simulink model "Batteries"  (R2026b)
settings: Solver=VariableStepAuto
undefined symbols (not defined in the file or in its folder): battery_builder_rtmsupport, gcbh
libraries: Batteries_lib x10
settings Model: Creator=andrei  LastModifiedBy=andrei

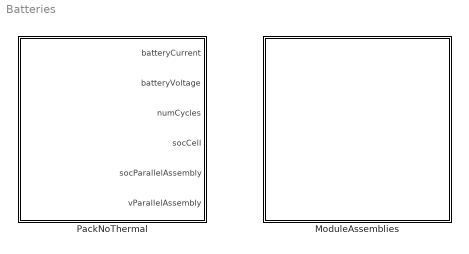
== system Batteries ==
  ModuleAssemblies : Subsystem
  PackNoThermal : Subsystem  LoadFcn=battery_builder_rtmsupport('loadfcn',gcbh);
      settings: CopyFcn=battery_builder_rtmsupport('copyfcn',gcbh);  PreCopyFcn=battery_builder_rtmsupport('precopyfcn',gcbh);  PreDeleteFcn=battery_builder_rtmsupport('predeletefcn',gcbh);  PortSchema="{\"entries\":[{\"content\":{\"sides\":[{\"content\":{\"connectorIds\":[\"LConn1\"]},\"type\":\"ConnectorPlacement.EquallySpacedRectSide\",\"uuid\":\"dcefa4cb-5347-4db9-a4bb-b951e3d91390\"},{\"content\":{\"connectorIds\":[\"RConn1\"],\"side\":\"RIGHT\"},\"type\":\"ConnectorPlacement.EquallySpacedRectSide\",\"uuid\":\"aeb17dee-f2a5-4d63-887b-6da27d52d7b7\"},{\"content\":{\"side\":\"TOP\"},\"type\":\"ConnectorPlacement.EquallySpacedRectSide\",\"uuid\":\"cfb96706-c05e-4745-bfe0-c570812fde5c\"},{\"content\":{\"connectorIds\":[\"Out1\",\"Out2\",\"Out3\",\"Out4\",\"Out5\",\"Out6\"],\"side\":\"BOTTOM\"},\"type\":\"ConnectorPlacement.EquallySpacedRectSide\",\"uuid\":\"433bdf42-6f85-4686-85d7-f0461854e351\"}]},\"type\":\"ConnectorPlacement.EquallySpacedConnector\",\"uuid\":\"fe86a992-77e4-407d-ab55-7155ee49e73e\"}],\"packageUris\":[\"http://schema.mathworks.com/mf0/Connector/R2020b\"],\"version\":\"1.0\"}"
      mask Display: image('$imagefile')

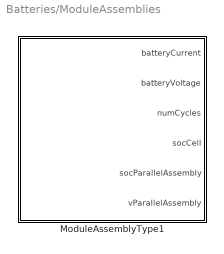
== system Batteries/ModuleAssemblies ==
  ModuleAssemblyType1 : Subsystem  LoadFcn=battery_builder_rtmsupport('loadfcn',gcbh);
      settings: CopyFcn=battery_builder_rtmsupport('copyfcn',gcbh);  PreCopyFcn=battery_builder_rtmsupport('precopyfcn',gcbh);  PreDeleteFcn=battery_builder_rtmsupport('predeletefcn',gcbh);  PortSchema="{\"entries\":[{\"content\":{\"sides\":[{\"content\":{\"connectorIds\":[\"LConn1\"]},\"type\":\"ConnectorPlacement.EquallySpacedRectSide\",\"uuid\":\"dcefa4cb-5347-4db9-a4bb-b951e3d91390\"},{\"content\":{\"connectorIds\":[\"RConn1\"],\"side\":\"RIGHT\"},\"type\":\"ConnectorPlacement.EquallySpacedRectSide\",\"uuid\":\"aeb17dee-f2a5-4d63-887b-6da27d52d7b7\"},{\"content\":{\"side\":\"TOP\"},\"type\":\"ConnectorPlacement.EquallySpacedRectSide\",\"uuid\":\"cfb96706-c05e-4745-bfe0-c570812fde5c\"},{\"content\":{\"connectorIds\":[\"Out1\",\"Out2\",\"Out3\",\"Out4\",\"Out5\",\"Out6\"],\"side\":\"BOTTOM\"},\"type\":\"ConnectorPlacement.EquallySpacedRectSide\",\"uuid\":\"431ac705-a0e6-4cbc-989d-1f8ff93ff9b4\"}]},\"type\":\"ConnectorPlacement.EquallySpacedConnector\",\"uuid\":\"fe86a992-77e4-407d-ab55-7155ee49e73e\"}],\"packageUris\":[\"http://schema.mathworks.com/mf0/Connector/R2020b\"],\"version\":\"1.0\"}"
      mask Display: image('$imagefile')

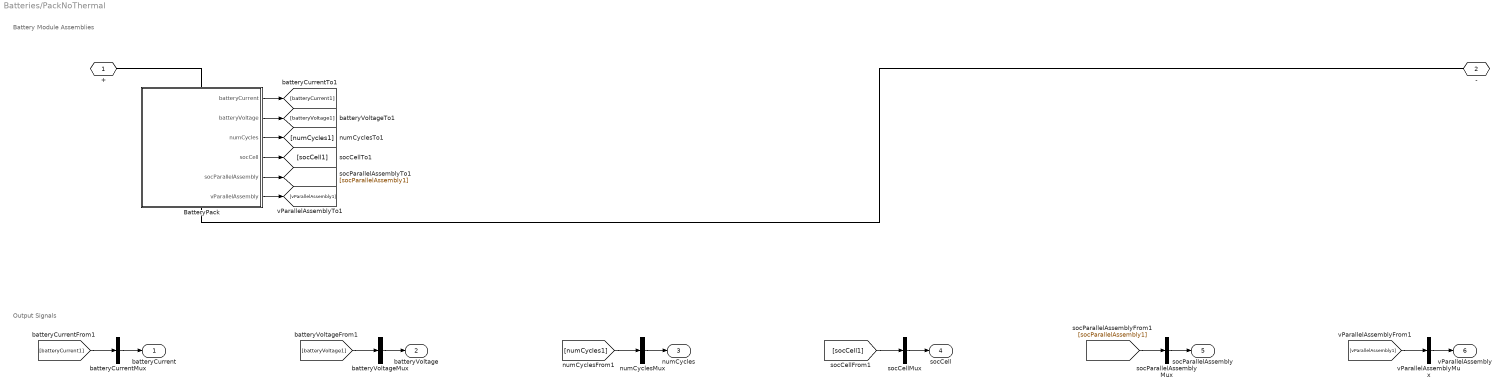
== system Batteries/PackNoThermal ==
  note: Battery Module Assemblies
  note: Output Signals
  BatteryPack : Subsystem  LoadFcn=battery_builder_rtmsupport('loadfcn',gcbh);
      settings: CopyFcn=battery_builder_rtmsupport('copyfcn',gcbh);  PreCopyFcn=battery_builder_rtmsupport('precopyfcn',gcbh);  PreDeleteFcn=battery_builder_rtmsupport('predeletefcn',gcbh);  PortSchema="{\"entries\":[{\"content\":{\"sides\":[{\"content\":{\"connectorIds\":[\"LConn1\"]},\"type\":\"ConnectorPlacement.EquallySpacedRectSide\",\"uuid\":\"dcefa4cb-5347-4db9-a4bb-b951e3d91390\"},{\"content\":{\"connectorIds\":[\"RConn1\"],\"side\":\"RIGHT\"},\"type\":\"ConnectorPlacement.EquallySpacedRectSide\",\"uuid\":\"aeb17dee-f2a5-4d63-887b-6da27d52d7b7\"},{\"content\":{\"side\":\"TOP\"},\"type\":\"ConnectorPlacement.EquallySpacedRectSide\",\"uuid\":\"cfb96706-c05e-4745-bfe0-c570812fde5c\"},{\"content\":{\"connectorIds\":[\"Out1\",\"Out2\",\"Out3\",\"Out4\",\"Out5\",\"Out6\"],\"side\":\"BOTTOM\"},\"type\":\"ConnectorPlacement.EquallySpacedRectSide\",\"uuid\":\"431ac705-a0e6-4cbc-989d-1f8ff93ff9b4\"}]},\"type\":\"ConnectorPlacement.EquallySpacedConnector\",\"uuid\":\"fe86a992-77e4-407d-ab55-7155ee49e73e\"}],\"packageUris\":[\"http://schema.mathworks.com/mf0/Connector/R2020b\"],\"version\":\"1.0\"}"
      mask Display: image('$imagefile')
  batteryCurrentMux : Mux  Inputs=1
  batteryVoltageMux : Mux  Inputs=1
  numCyclesMux : Mux  Inputs=1
  socCellMux : Mux  Inputs=1
  socParallelAssemblyMux : Mux  Inputs=1
  vParallelAssemblyMux : Mux  Inputs=1
  + : PMIOPort  Side=Left
  - : PMIOPort  Port=2  Side=Right
  batteryCurrent : Outport
  batteryVoltage : Outport  Port=2
  numCycles : Outport  Port=3
  socCell : Outport  Port=4
  socParallelAssembly : Outport  Port=5
  vParallelAssembly : Outport  Port=6
  wires:
  BatteryPack/1(batteryCurrent) -> [batteryCurrent1]
  batteryCurrentMux/1 -> batteryCurrent/1
  [batteryCurrent1] -> batteryCurrentMux/1
  BatteryPack/2(batteryVoltage) -> [batteryVoltage1]
  batteryVoltageMux/1 -> batteryVoltage/1
  [batteryVoltage1] -> batteryVoltageMux/1
  BatteryPack/3(numCycles) -> [numCycles1]
  numCyclesMux/1 -> numCycles/1
  [numCycles1] -> numCyclesMux/1
  BatteryPack/4(socCell) -> [socCell1]
  socCellMux/1 -> socCell/1
  [socCell1] -> socCellMux/1
  BatteryPack/5(socParallelAssembly) -> [socParallelAssembly1]
  socParallelAssemblyMux/1 -> socParallelAssembly/1
  [socParallelAssembly1] -> socParallelAssemblyMux/1
  BatteryPack/6(vParallelAssembly) -> [vParallelAssembly1]
  vParallelAssemblyMux/1 -> vParallelAssembly/1
  [vParallelAssembly1] -> vParallelAssemblyMux/1
  connections:
  BatteryPack/LConn1 -- +/RConn1
  BatteryPack/RConn1 -- -/RConn1

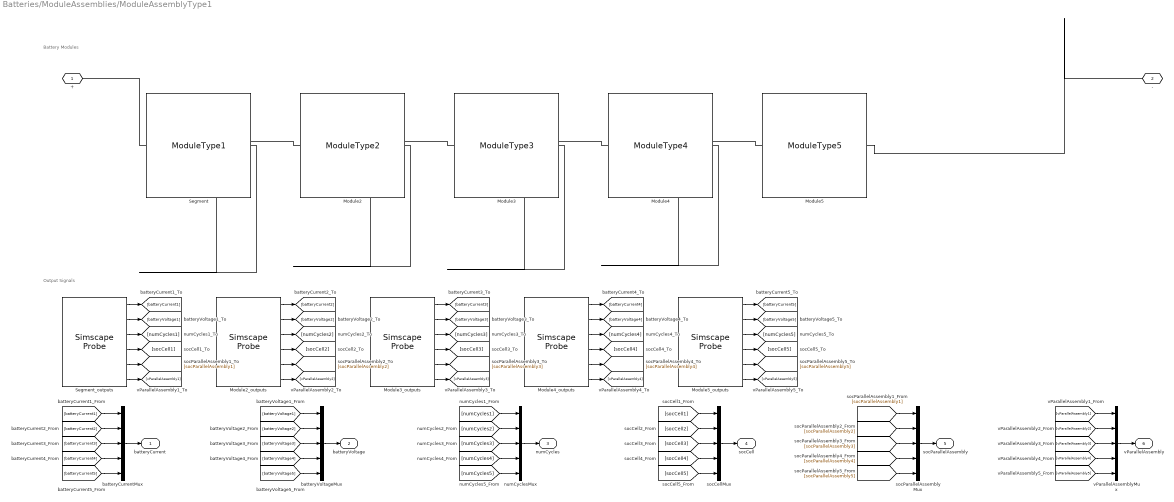
== system Batteries/ModuleAssemblies/ModuleAssemblyType1 ==
  note: Battery Modules
  note: Output Signals
  Module2 : Batteries_lib/Modules/ModuleType2  BatteryCapacityCell=27 A*hr  ExtrapolationMethodCell=simscape.enum.extrapolation.nearest  SOCBreakpointsCell=[0, .1, .25, .5, .75, .9, 1]  TemperatureBreakpointsCell=[278, 293, 313] K  OpenCircuitVoltageThermalCell=[3.49, 3.5, 3.51; 3.55, 3.57, 3.56; 3.62, 3.63, 3.64; 3.71, 3.71, 3.72; 3.91, 3.93, 3.94; 4.07, 4.08, 4.08; 4.19, 4.19, 4.19] V  VoltageRangeCell=[0, inf] V  ResistanceSOCBreakpointsCell=[0, .1, .25, .5, .75, .9, 1]  ResistanceTemperatureBreakpointsCell=[278, 293, 313] K  R0ThermalCell=[.0117, .0085, .009; .011, .0085, .009; .0114, .0087, .0092; .0107, .0082, .0088; .0107, .0083, .0091; .0113, .0085, .0089; .0116, .0085, .0089] Ohm  SimulationTemperatureCell=298.15 K  socCell_specify=off  socCell_priority=High  socCell=repmat(1, 75, 1)  socCell_nominal_specify=off  socCell_nominal_value=1  socCell_nominal_unit=1  batteryVoltage_specify=off  batteryVoltage_priority=None  batteryVoltage=repmat(0, 75, 1) V  batteryVoltage_nominal_specify=off  batteryVoltage_nominal_value=1  batteryVoltage_nominal_unit=V  batteryCurrent_specify=off  batteryCurrent_priority=None  batteryCurrent=repmat(0, 75, 1) A  batteryCurrent_nominal_specify=off  batteryCurrent_nominal_value=1  batteryCurrent_nominal_unit=A  numCycles_specify=off  numCycles_priority=High  numCycles=repmat(0, 75, 1)  numCycles_nominal_specify=off  numCycles_nominal_value=1  numCycles_nominal_unit=1  vParallelAssembly_specify=off  vParallelAssembly_priority=None  vParallelAssembly=repmat(0, 15, 1) V  vParallelAssembly_nominal_specify=off  vParallelAssembly_nominal_value=1  vParallelAssembly_nominal_unit=V  socParallelAssembly_specify=off  socParallelAssembly_priority=None  socParallelAssembly=repmat(1, 15, 1)  socParallelAssembly_nominal_specify=off  socParallelAssembly_nominal_value=1  socParallelAssembly_nominal_unit=1
  Module2_outputs : SimscapeProbe  BoundBlock=4  Variables="{\"batteryCurrent\":{\"Probing\":\"ON\"},\"batteryVoltage\":{\"Probing\":\"ON\"},\"numCycles\":{\"Probing\":\"ON\"},\"socCell\":{\"Probing\":\"ON\"},\"socParallelAssembly\":{\"Probing\":\"ON\"},\"vParallelAssembly\":{\"Probing\":\"ON\"}}"
  Module3 : Batteries_lib/Modules/ModuleType3  BatteryCapacityCell=27 A*hr  ExtrapolationMethodCell=simscape.enum.extrapolation.nearest  SOCBreakpointsCell=[0, .1, .25, .5, .75, .9, 1]  TemperatureBreakpointsCell=[278, 293, 313] K  OpenCircuitVoltageThermalCell=[3.49, 3.5, 3.51; 3.55, 3.57, 3.56; 3.62, 3.63, 3.64; 3.71, 3.71, 3.72; 3.91, 3.93, 3.94; 4.07, 4.08, 4.08; 4.19, 4.19, 4.19] V  VoltageRangeCell=[0, inf] V  ResistanceSOCBreakpointsCell=[0, .1, .25, .5, .75, .9, 1]  ResistanceTemperatureBreakpointsCell=[278, 293, 313] K  R0ThermalCell=[.0117, .0085, .009; .011, .0085, .009; .0114, .0087, .0092; .0107, .0082, .0088; .0107, .0083, .0091; .0113, .0085, .0089; .0116, .0085, .0089] Ohm  SimulationTemperatureCell=298.15 K  socCell_specify=off  socCell_priority=High  socCell=repmat(1, 75, 1)  socCell_nominal_specify=off  socCell_nominal_value=1  socCell_nominal_unit=1  batteryVoltage_specify=off  batteryVoltage_priority=None  batteryVoltage=repmat(0, 75, 1) V  batteryVoltage_nominal_specify=off  batteryVoltage_nominal_value=1  batteryVoltage_nominal_unit=V  batteryCurrent_specify=off  batteryCurrent_priority=None  batteryCurrent=repmat(0, 75, 1) A  batteryCurrent_nominal_specify=off  batteryCurrent_nominal_value=1  batteryCurrent_nominal_unit=A  numCycles_specify=off  numCycles_priority=High  numCycles=repmat(0, 75, 1)  numCycles_nominal_specify=off  numCycles_nominal_value=1  numCycles_nominal_unit=1  vParallelAssembly_specify=off  vParallelAssembly_priority=None  vParallelAssembly=repmat(0, 15, 1) V  vParallelAssembly_nominal_specify=off  vParallelAssembly_nominal_value=1  vParallelAssembly_nominal_unit=V  socParallelAssembly_specify=off  socParallelAssembly_priority=None  socParallelAssembly=repmat(1, 15, 1)  socParallelAssembly_nominal_specify=off  socParallelAssembly_nominal_value=1  socParallelAssembly_nominal_unit=1
  Module3_outputs : SimscapeProbe  BoundBlock=5  Variables="{\"batteryCurrent\":{\"Probing\":\"ON\"},\"batteryVoltage\":{\"Probing\":\"ON\"},\"numCycles\":{\"Probing\":\"ON\"},\"socCell\":{\"Probing\":\"ON\"},\"socParallelAssembly\":{\"Probing\":\"ON\"},\"vParallelAssembly\":{\"Probing\":\"ON\"}}"
  Module4 : Batteries_lib/Modules/ModuleType4  BatteryCapacityCell=27 A*hr  ExtrapolationMethodCell=simscape.enum.extrapolation.nearest  SOCBreakpointsCell=[0, .1, .25, .5, .75, .9, 1]  TemperatureBreakpointsCell=[278, 293, 313] K  OpenCircuitVoltageThermalCell=[3.49, 3.5, 3.51; 3.55, 3.57, 3.56; 3.62, 3.63, 3.64; 3.71, 3.71, 3.72; 3.91, 3.93, 3.94; 4.07, 4.08, 4.08; 4.19, 4.19, 4.19] V  VoltageRangeCell=[0, inf] V  ResistanceSOCBreakpointsCell=[0, .1, .25, .5, .75, .9, 1]  ResistanceTemperatureBreakpointsCell=[278, 293, 313] K  R0ThermalCell=[.0117, .0085, .009; .011, .0085, .009; .0114, .0087, .0092; .0107, .0082, .0088; .0107, .0083, .0091; .0113, .0085, .0089; .0116, .0085, .0089] Ohm  SimulationTemperatureCell=298.15 K  socCell_specify=off  socCell_priority=High  socCell=repmat(1, 75, 1)  socCell_nominal_specify=off  socCell_nominal_value=1  socCell_nominal_unit=1  batteryVoltage_specify=off  batteryVoltage_priority=None  batteryVoltage=repmat(0, 75, 1) V  batteryVoltage_nominal_specify=off  batteryVoltage_nominal_value=1  batteryVoltage_nominal_unit=V  batteryCurrent_specify=off  batteryCurrent_priority=None  batteryCurrent=repmat(0, 75, 1) A  batteryCurrent_nominal_specify=off  batteryCurrent_nominal_value=1  batteryCurrent_nominal_unit=A  numCycles_specify=off  numCycles_priority=High  numCycles=repmat(0, 75, 1)  numCycles_nominal_specify=off  numCycles_nominal_value=1  numCycles_nominal_unit=1  vParallelAssembly_specify=off  vParallelAssembly_priority=None  vParallelAssembly=repmat(0, 15, 1) V  vParallelAssembly_nominal_specify=off  vParallelAssembly_nominal_value=1  vParallelAssembly_nominal_unit=V  socParallelAssembly_specify=off  socParallelAssembly_priority=None  socParallelAssembly=repmat(1, 15, 1)  socParallelAssembly_nominal_specify=off  socParallelAssembly_nominal_value=1  socParallelAssembly_nominal_unit=1
  Module4_outputs : SimscapeProbe  BoundBlock=6  Variables="{\"batteryCurrent\":{\"Probing\":\"ON\"},\"batteryVoltage\":{\"Probing\":\"ON\"},\"numCycles\":{\"Probing\":\"ON\"},\"socCell\":{\"Probing\":\"ON\"},\"socParallelAssembly\":{\"Probing\":\"ON\"},\"vParallelAssembly\":{\"Probing\":\"ON\"}}"
  Module5 : Batteries_lib/Modules/ModuleType5  BatteryCapacityCell=27 A*hr  ExtrapolationMethodCell=simscape.enum.extrapolation.nearest  SOCBreakpointsCell=[0, .1, .25, .5, .75, .9, 1]  TemperatureBreakpointsCell=[278, 293, 313] K  OpenCircuitVoltageThermalCell=[3.49, 3.5, 3.51; 3.55, 3.57, 3.56; 3.62, 3.63, 3.64; 3.71, 3.71, 3.72; 3.91, 3.93, 3.94; 4.07, 4.08, 4.08; 4.19, 4.19, 4.19] V  VoltageRangeCell=[0, inf] V  ResistanceSOCBreakpointsCell=[0, .1, .25, .5, .75, .9, 1]  ResistanceTemperatureBreakpointsCell=[278, 293, 313] K  R0ThermalCell=[.0117, .0085, .009; .011, .0085, .009; .0114, .0087, .0092; .0107, .0082, .0088; .0107, .0083, .0091; .0113, .0085, .0089; .0116, .0085, .0089] Ohm  SimulationTemperatureCell=298.15 K  socCell_specify=off  socCell_priority=High  socCell=repmat(1, 75, 1)  socCell_nominal_specify=off  socCell_nominal_value=1  socCell_nominal_unit=1  batteryVoltage_specify=off  batteryVoltage_priority=None  batteryVoltage=repmat(0, 75, 1) V  batteryVoltage_nominal_specify=off  batteryVoltage_nominal_value=1  batteryVoltage_nominal_unit=V  batteryCurrent_specify=off  batteryCurrent_priority=None  batteryCurrent=repmat(0, 75, 1) A  batteryCurrent_nominal_specify=off  batteryCurrent_nominal_value=1  batteryCurrent_nominal_unit=A  numCycles_specify=off  numCycles_priority=High  numCycles=repmat(0, 75, 1)  numCycles_nominal_specify=off  numCycles_nominal_value=1  numCycles_nominal_unit=1  vParallelAssembly_specify=off  vParallelAssembly_priority=None  vParallelAssembly=repmat(0, 15, 1) V  vParallelAssembly_nominal_specify=off  vParallelAssembly_nominal_value=1  vParallelAssembly_nominal_unit=V  socParallelAssembly_specify=off  socParallelAssembly_priority=None  socParallelAssembly=repmat(1, 15, 1)  socParallelAssembly_nominal_specify=off  socParallelAssembly_nominal_value=1  socParallelAssembly_nominal_unit=1
  Module5_outputs : SimscapeProbe  BoundBlock=7  Variables="{\"batteryCurrent\":{\"Probing\":\"ON\"},\"batteryVoltage\":{\"Probing\":\"ON\"},\"numCycles\":{\"Probing\":\"ON\"},\"socCell\":{\"Probing\":\"ON\"},\"socParallelAssembly\":{\"Probing\":\"ON\"},\"vParallelAssembly\":{\"Probing\":\"ON\"}}"
  Segment : Batteries_lib/Modules/ModuleType1  BatteryCapacityCell=27 A*hr  ExtrapolationMethodCell=simscape.enum.extrapolation.nearest  SOCBreakpointsCell=[0, .1, .25, .5, .75, .9, 1]  TemperatureBreakpointsCell=[278, 293, 313] K  OpenCircuitVoltageThermalCell=[3.49, 3.5, 3.51; 3.55, 3.57, 3.56; 3.62, 3.63, 3.64; 3.71, 3.71, 3.72; 3.91, 3.93, 3.94; 4.07, 4.08, 4.08; 4.19, 4.19, 4.19] V  VoltageRangeCell=[0, inf] V  ResistanceSOCBreakpointsCell=[0, .1, .25, .5, .75, .9, 1]  ResistanceTemperatureBreakpointsCell=[278, 293, 313] K  R0ThermalCell=[.0117, .0085, .009; .011, .0085, .009; .0114, .0087, .0092; .0107, .0082, .0088; .0107, .0083, .0091; .0113, .0085, .0089; .0116, .0085, .0089] Ohm  SimulationTemperatureCell=298.15 K  socCell_specify=off  socCell_priority=High  socCell=repmat(1, 75, 1)  socCell_nominal_specify=off  socCell_nominal_value=1  socCell_nominal_unit=1  batteryVoltage_specify=off  batteryVoltage_priority=None  batteryVoltage=repmat(0, 75, 1) V  batteryVoltage_nominal_specify=off  batteryVoltage_nominal_value=1  batteryVoltage_nominal_unit=V  batteryCurrent_specify=off  batteryCurrent_priority=None  batteryCurrent=repmat(0, 75, 1) A  batteryCurrent_nominal_specify=off  batteryCurrent_nominal_value=1  batteryCurrent_nominal_unit=A  numCycles_specify=off  numCycles_priority=High  numCycles=repmat(0, 75, 1)  numCycles_nominal_specify=off  numCycles_nominal_value=1  numCycles_nominal_unit=1  vParallelAssembly_specify=off  vParallelAssembly_priority=None  vParallelAssembly=repmat(0, 15, 1) V  vParallelAssembly_nominal_specify=off  vParallelAssembly_nominal_value=1  vParallelAssembly_nominal_unit=V  socParallelAssembly_specify=off  socParallelAssembly_priority=None  socParallelAssembly=repmat(1, 15, 1)  socParallelAssembly_nominal_specify=off  socParallelAssembly_nominal_value=1  socParallelAssembly_nominal_unit=1
  Segment_outputs : SimscapeProbe  BoundBlock=3  Variables="{\"batteryCurrent\":{\"Probing\":\"ON\"},\"batteryVoltage\":{\"Probing\":\"ON\"},\"numCycles\":{\"Probing\":\"ON\"},\"socCell\":{\"Probing\":\"ON\"},\"socParallelAssembly\":{\"Probing\":\"ON\"},\"vParallelAssembly\":{\"Probing\":\"ON\"}}"
  batteryCurrentMux : Mux  Inputs=5
  batteryVoltageMux : Mux  Inputs=5
  numCyclesMux : Mux  Inputs=5
  socCellMux : Mux  Inputs=5
  socParallelAssemblyMux : Mux  Inputs=5
  vParallelAssemblyMux : Mux  Inputs=5
  + : PMIOPort  Side=Left
  - : PMIOPort  Port=2  Side=Right
  batteryCurrent : Outport
  batteryVoltage : Outport  Port=2
  numCycles : Outport  Port=3
  socCell : Outport  Port=4
  socParallelAssembly : Outport  Port=5
  vParallelAssembly : Outport  Port=6
  wires:
  Segment_outputs/1 -> [batteryCurrent1]
  batteryCurrentMux/1 -> batteryCurrent/1
  [batteryCurrent1] -> batteryCurrentMux/1
  Segment_outputs/2 -> [batteryVoltage1]
  batteryVoltageMux/1 -> batteryVoltage/1
  [batteryVoltage1] -> batteryVoltageMux/1
  Segment_outputs/3 -> [numCycles1]
  numCyclesMux/1 -> numCycles/1
  [numCycles1] -> numCyclesMux/1
  Segment_outputs/4 -> [socCell1]
  socCellMux/1 -> socCell/1
  [socCell1] -> socCellMux/1
  Segment_outputs/5 -> [socParallelAssembly1]
  socParallelAssemblyMux/1 -> socParallelAssembly/1
  [socParallelAssembly1] -> socParallelAssemblyMux/1
  Segment_outputs/6 -> [vParallelAssembly1]
  vParallelAssemblyMux/1 -> vParallelAssembly/1
  [vParallelAssembly1] -> vParallelAssemblyMux/1
  Module2_outputs/1 -> [batteryCurrent2]
  [batteryCurrent2] -> batteryCurrentMux/2
  Module2_outputs/2 -> [batteryVoltage2]
  [batteryVoltage2] -> batteryVoltageMux/2
  Module2_outputs/3 -> [numCycles2]
  [numCycles2] -> numCyclesMux/2
  Module2_outputs/4 -> [socCell2]
  [socCell2] -> socCellMux/2
  Module2_outputs/5 -> [socParallelAssembly2]
  [socParallelAssembly2] -> socParallelAssemblyMux/2
  Module2_outputs/6 -> [vParallelAssembly2]
  [vParallelAssembly2] -> vParallelAssemblyMux/2
  Module3_outputs/1 -> [batteryCurrent3]
  [batteryCurrent3] -> batteryCurrentMux/3
  Module3_outputs/2 -> [batteryVoltage3]
  [batteryVoltage3] -> batteryVoltageMux/3
  Module3_outputs/3 -> [numCycles3]
  [numCycles3] -> numCyclesMux/3
  Module3_outputs/4 -> [socCell3]
  [socCell3] -> socCellMux/3
  Module3_outputs/5 -> [socParallelAssembly3]
  [socParallelAssembly3] -> socParallelAssemblyMux/3
  Module3_outputs/6 -> [vParallelAssembly3]
  [vParallelAssembly3] -> vParallelAssemblyMux/3
  Module4_outputs/1 -> [batteryCurrent4]
  [batteryCurrent4] -> batteryCurrentMux/4
  Module4_outputs/2 -> [batteryVoltage4]
  [batteryVoltage4] -> batteryVoltageMux/4
  Module4_outputs/3 -> [numCycles4]
  [numCycles4] -> numCyclesMux/4
  Module4_outputs/4 -> [socCell4]
  [socCell4] -> socCellMux/4
  Module4_outputs/5 -> [socParallelAssembly4]
  [socParallelAssembly4] -> socParallelAssemblyMux/4
  Module4_outputs/6 -> [vParallelAssembly4]
  [vParallelAssembly4] -> vParallelAssemblyMux/4
  Module5_outputs/1 -> [batteryCurrent5]
  [batteryCurrent5] -> batteryCurrentMux/5
  Module5_outputs/2 -> [batteryVoltage5]
  [batteryVoltage5] -> batteryVoltageMux/5
  Module5_outputs/3 -> [numCycles5]
  [numCycles5] -> numCyclesMux/5
  Module5_outputs/4 -> [socCell5]
  [socCell5] -> socCellMux/5
  Module5_outputs/5 -> [socParallelAssembly5]
  [socParallelAssembly5] -> socParallelAssemblyMux/5
  Module5_outputs/6 -> [vParallelAssembly5]
  [vParallelAssembly5] -> vParallelAssemblyMux/5
  connections:
  Module2/LConn1 -- Segment/RConn1
  Module3/LConn1 -- Module2/RConn1
  Module4/LConn1 -- Module3/RConn1
  Module5/LConn1 -- Module4/RConn1
  Segment/LConn1 -- +/RConn1
  Module5/RConn1 -- -/RConn1

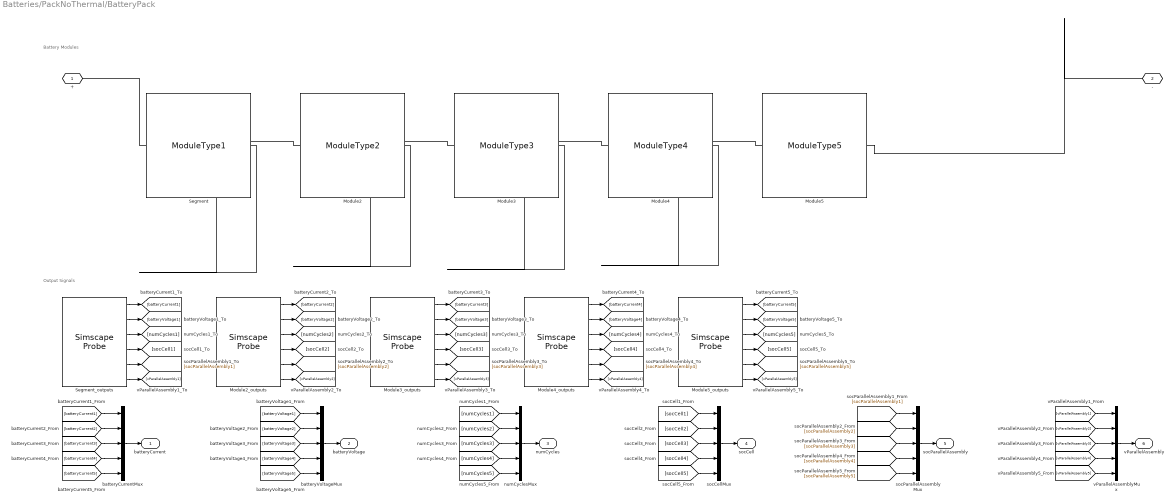
== system Batteries/PackNoThermal/BatteryPack ==
  note: Output Signals
  note: Battery Modules
  Module2 : Batteries_lib/Modules/ModuleType2  BatteryCapacityCell=BatteryPack.Segment.BatteryCapacityCell A*hr  ExtrapolationMethodCell=simscape.enum.extrapolation.nearest  SOCBreakpointsCell=BatteryPack.Segment.SOCBreakpointsCell  TemperatureBreakpointsCell=BatteryPack.Segment.TemperatureBreakpointsCell K  OpenCircuitVoltageThermalCell=BatteryPack.Segment.OpenCircuitVoltageThermalCell V  VoltageRangeCell=BatteryPack.Segment.VoltageRangeCell V  ResistanceSOCBreakpointsCell=BatteryPack.Segment.ResistanceSOCBreakpointsCell  ResistanceTemperatureBreakpointsCell=BatteryPack.Segment.ResistanceTemperatureBreakpointsCell K  R0ThermalCell=BatteryPack.Segment.R0ThermalCell Ohm  SimulationTemperatureCell=BatteryPack.Segment.SimulationTemperatureCell K  socCell_specify=on  socCell_priority=High  socCell=[1;1;1;1;1;1;1;1;1;1;1;1;1;1;1;1;1;1;1;1;1;1;1;1;1;1;1;1;1;1;1;1;1;1;1;1;1;1;1;1;1;1;1;1;1;1;1;1;1;1;1;1;1;1;1;1;1;1;1;1;1;1;1;1;1;1;1;1;1;1;1;1;1;1;1]  socCell_nominal_specify=off  socCell_nominal_value=1  socCell_nominal_unit=1  batteryVoltage_specify=on  batteryVoltage_priority=None  batteryVoltage=[0;0;0;0;0;0;0;0;0;0;0;0;0;0;0;0;0;0;0;0;0;0;0;0;0;0;0;0;0;0;0;0;0;0;0;0;0;0;0;0;0;0;0;0;0;0;0;0;0;0;0;0;0;0;0;0;0;0;0;0;0;0;0;0;0;0;0;0;0;0;0;0;0;0;0] V  batteryVoltage_nominal_specify=off  batteryVoltage_nominal_value=1  batteryVoltage_nominal_unit=V  batteryCurrent_specify=on  batteryCurrent_priority=None  batteryCurrent=[0;0;0;0;0;0;0;0;0;0;0;0;0;0;0;0;0;0;0;0;0;0;0;0;0;0;0;0;0;0;0;0;0;0;0;0;0;0;0;0;0;0;0;0;0;0;0;0;0;0;0;0;0;0;0;0;0;0;0;0;0;0;0;0;0;0;0;0;0;0;0;0;0;0;0] A  batteryCurrent_nominal_specify=off  batteryCurrent_nominal_value=1  batteryCurrent_nominal_unit=A  numCycles_specify=on  numCycles_priority=High  numCycles=[0;0;0;0;0;0;0;0;0;0;0;0;0;0;0;0;0;0;0;0;0;0;0;0;0;0;0;0;0;0;0;0;0;0;0;0;0;0;0;0;0;0;0;0;0;0;0;0;0;0;0;0;0;0;0;0;0;0;0;0;0;0;0;0;0;0;0;0;0;0;0;0;0;0;0]  numCycles_nominal_specify=off  numCycles_nominal_value=1  numCycles_nominal_unit=1  vParallelAssembly_specify=on  vParallelAssembly_priority=None  vParallelAssembly=[0;0;0;0;0;0;0;0;0;0;0;0;0;0;0] V  vParallelAssembly_nominal_specify=off  vParallelAssembly_nominal_value=1  vParallelAssembly_nominal_unit=V  socParallelAssembly_specify=on  socParallelAssembly_priority=None  socParallelAssembly=[1;1;1;1;1;1;1;1;1;1;1;1;1;1;1]  socParallelAssembly_nominal_specify=off  socParallelAssembly_nominal_value=1  socParallelAssembly_nominal_unit=1
  Module2_outputs : SimscapeProbe  BoundBlock=91  Variables="{\"batteryCurrent\":{\"Probing\":\"ON\"},\"batteryVoltage\":{\"Probing\":\"ON\"},\"numCycles\":{\"Probing\":\"ON\"},\"socCell\":{\"Probing\":\"ON\"},\"socParallelAssembly\":{\"Probing\":\"ON\"},\"vParallelAssembly\":{\"Probing\":\"ON\"}}"
  Module3 : Batteries_lib/Modules/ModuleType3  BatteryCapacityCell=BatteryPack.Segment.BatteryCapacityCell A*hr  ExtrapolationMethodCell=simscape.enum.extrapolation.nearest  SOCBreakpointsCell=BatteryPack.Segment.SOCBreakpointsCell  TemperatureBreakpointsCell=BatteryPack.Segment.TemperatureBreakpointsCell K  OpenCircuitVoltageThermalCell=BatteryPack.Segment.OpenCircuitVoltageThermalCell V  VoltageRangeCell=BatteryPack.Segment.VoltageRangeCell V  ResistanceSOCBreakpointsCell=BatteryPack.Segment.ResistanceSOCBreakpointsCell  ResistanceTemperatureBreakpointsCell=BatteryPack.Segment.ResistanceTemperatureBreakpointsCell K  R0ThermalCell=BatteryPack.Segment.R0ThermalCell Ohm  SimulationTemperatureCell=BatteryPack.Segment.SimulationTemperatureCell K  socCell_specify=on  socCell_priority=High  socCell=[1;1;1;1;1;1;1;1;1;1;1;1;1;1;1;1;1;1;1;1;1;1;1;1;1;1;1;1;1;1;1;1;1;1;1;1;1;1;1;1;1;1;1;1;1;1;1;1;1;1;1;1;1;1;1;1;1;1;1;1;1;1;1;1;1;1;1;1;1;1;1;1;1;1;1]  socCell_nominal_specify=off  socCell_nominal_value=1  socCell_nominal_unit=1  batteryVoltage_specify=on  batteryVoltage_priority=None  batteryVoltage=[0;0;0;0;0;0;0;0;0;0;0;0;0;0;0;0;0;0;0;0;0;0;0;0;0;0;0;0;0;0;0;0;0;0;0;0;0;0;0;0;0;0;0;0;0;0;0;0;0;0;0;0;0;0;0;0;0;0;0;0;0;0;0;0;0;0;0;0;0;0;0;0;0;0;0] V  batteryVoltage_nominal_specify=off  batteryVoltage_nominal_value=1  batteryVoltage_nominal_unit=V  batteryCurrent_specify=on  batteryCurrent_priority=None  batteryCurrent=[0;0;0;0;0;0;0;0;0;0;0;0;0;0;0;0;0;0;0;0;0;0;0;0;0;0;0;0;0;0;0;0;0;0;0;0;0;0;0;0;0;0;0;0;0;0;0;0;0;0;0;0;0;0;0;0;0;0;0;0;0;0;0;0;0;0;0;0;0;0;0;0;0;0;0] A  batteryCurrent_nominal_specify=off  batteryCurrent_nominal_value=1  batteryCurrent_nominal_unit=A  numCycles_specify=on  numCycles_priority=High  numCycles=[0;0;0;0;0;0;0;0;0;0;0;0;0;0;0;0;0;0;0;0;0;0;0;0;0;0;0;0;0;0;0;0;0;0;0;0;0;0;0;0;0;0;0;0;0;0;0;0;0;0;0;0;0;0;0;0;0;0;0;0;0;0;0;0;0;0;0;0;0;0;0;0;0;0;0]  numCycles_nominal_specify=off  numCycles_nominal_value=1  numCycles_nominal_unit=1  vParallelAssembly_specify=on  vParallelAssembly_priority=None  vParallelAssembly=[0;0;0;0;0;0;0;0;0;0;0;0;0;0;0] V  vParallelAssembly_nominal_specify=off  vParallelAssembly_nominal_value=1  vParallelAssembly_nominal_unit=V  socParallelAssembly_specify=on  socParallelAssembly_priority=None  socParallelAssembly=[1;1;1;1;1;1;1;1;1;1;1;1;1;1;1]  socParallelAssembly_nominal_specify=off  socParallelAssembly_nominal_value=1  socParallelAssembly_nominal_unit=1
  Module3_outputs : SimscapeProbe  BoundBlock=93  Variables="{\"batteryCurrent\":{\"Probing\":\"ON\"},\"batteryVoltage\":{\"Probing\":\"ON\"},\"numCycles\":{\"Probing\":\"ON\"},\"socCell\":{\"Probing\":\"ON\"},\"socParallelAssembly\":{\"Probing\":\"ON\"},\"vParallelAssembly\":{\"Probing\":\"ON\"}}"
  Module4 : Batteries_lib/Modules/ModuleType4  BatteryCapacityCell=BatteryPack.Segment.BatteryCapacityCell A*hr  ExtrapolationMethodCell=simscape.enum.extrapolation.nearest  SOCBreakpointsCell=BatteryPack.Segment.SOCBreakpointsCell  TemperatureBreakpointsCell=BatteryPack.Segment.TemperatureBreakpointsCell K  OpenCircuitVoltageThermalCell=BatteryPack.Segment.OpenCircuitVoltageThermalCell V  VoltageRangeCell=BatteryPack.Segment.VoltageRangeCell V  ResistanceSOCBreakpointsCell=BatteryPack.Segment.ResistanceSOCBreakpointsCell  ResistanceTemperatureBreakpointsCell=BatteryPack.Segment.ResistanceTemperatureBreakpointsCell K  R0ThermalCell=BatteryPack.Segment.R0ThermalCell Ohm  SimulationTemperatureCell=BatteryPack.Segment.SimulationTemperatureCell K  socCell_specify=on  socCell_priority=High  socCell=[1;1;1;1;1;1;1;1;1;1;1;1;1;1;1;1;1;1;1;1;1;1;1;1;1;1;1;1;1;1;1;1;1;1;1;1;1;1;1;1;1;1;1;1;1;1;1;1;1;1;1;1;1;1;1;1;1;1;1;1;1;1;1;1;1;1;1;1;1;1;1;1;1;1;1]  socCell_nominal_specify=off  socCell_nominal_value=1  socCell_nominal_unit=1  batteryVoltage_specify=on  batteryVoltage_priority=None  batteryVoltage=[0;0;0;0;0;0;0;0;0;0;0;0;0;0;0;0;0;0;0;0;0;0;0;0;0;0;0;0;0;0;0;0;0;0;0;0;0;0;0;0;0;0;0;0;0;0;0;0;0;0;0;0;0;0;0;0;0;0;0;0;0;0;0;0;0;0;0;0;0;0;0;0;0;0;0] V  batteryVoltage_nominal_specify=off  batteryVoltage_nominal_value=1  batteryVoltage_nominal_unit=V  batteryCurrent_specify=on  batteryCurrent_priority=None  batteryCurrent=[0;0;0;0;0;0;0;0;0;0;0;0;0;0;0;0;0;0;0;0;0;0;0;0;0;0;0;0;0;0;0;0;0;0;0;0;0;0;0;0;0;0;0;0;0;0;0;0;0;0;0;0;0;0;0;0;0;0;0;0;0;0;0;0;0;0;0;0;0;0;0;0;0;0;0] A  batteryCurrent_nominal_specify=off  batteryCurrent_nominal_value=1  batteryCurrent_nominal_unit=A  numCycles_specify=on  numCycles_priority=High  numCycles=[0;0;0;0;0;0;0;0;0;0;0;0;0;0;0;0;0;0;0;0;0;0;0;0;0;0;0;0;0;0;0;0;0;0;0;0;0;0;0;0;0;0;0;0;0;0;0;0;0;0;0;0;0;0;0;0;0;0;0;0;0;0;0;0;0;0;0;0;0;0;0;0;0;0;0]  numCycles_nominal_specify=off  numCycles_nominal_value=1  numCycles_nominal_unit=1  vParallelAssembly_specify=on  vParallelAssembly_priority=None  vParallelAssembly=[0;0;0;0;0;0;0;0;0;0;0;0;0;0;0] V  vParallelAssembly_nominal_specify=off  vParallelAssembly_nominal_value=1  vParallelAssembly_nominal_unit=V  socParallelAssembly_specify=on  socParallelAssembly_priority=None  socParallelAssembly=[1;1;1;1;1;1;1;1;1;1;1;1;1;1;1]  socParallelAssembly_nominal_specify=off  socParallelAssembly_nominal_value=1  socParallelAssembly_nominal_unit=1
  Module4_outputs : SimscapeProbe  BoundBlock=95  Variables="{\"batteryCurrent\":{\"Probing\":\"ON\"},\"batteryVoltage\":{\"Probing\":\"ON\"},\"numCycles\":{\"Probing\":\"ON\"},\"socCell\":{\"Probing\":\"ON\"},\"socParallelAssembly\":{\"Probing\":\"ON\"},\"vParallelAssembly\":{\"Probing\":\"ON\"}}"
  Module5 : Batteries_lib/Modules/ModuleType5  BatteryCapacityCell=BatteryPack.Segment.BatteryCapacityCell A*hr  ExtrapolationMethodCell=simscape.enum.extrapolation.nearest  SOCBreakpointsCell=BatteryPack.Segment.SOCBreakpointsCell  TemperatureBreakpointsCell=BatteryPack.Segment.TemperatureBreakpointsCell K  OpenCircuitVoltageThermalCell=BatteryPack.Segment.OpenCircuitVoltageThermalCell V  VoltageRangeCell=BatteryPack.Segment.VoltageRangeCell V  ResistanceSOCBreakpointsCell=BatteryPack.Segment.ResistanceSOCBreakpointsCell  ResistanceTemperatureBreakpointsCell=BatteryPack.Segment.ResistanceTemperatureBreakpointsCell K  R0ThermalCell=BatteryPack.Segment.R0ThermalCell Ohm  SimulationTemperatureCell=BatteryPack.Segment.SimulationTemperatureCell K  socCell_specify=on  socCell_priority=High  socCell=[1;1;1;1;1;1;1;1;1;1;1;1;1;1;1;1;1;1;1;1;1;1;1;1;1;1;1;1;1;1;1;1;1;1;1;1;1;1;1;1;1;1;1;1;1;1;1;1;1;1;1;1;1;1;1;1;1;1;1;1;1;1;1;1;1;1;1;1;1;1;1;1;1;1;1]  socCell_nominal_specify=off  socCell_nominal_value=1  socCell_nominal_unit=1  batteryVoltage_specify=on  batteryVoltage_priority=None  batteryVoltage=[0;0;0;0;0;0;0;0;0;0;0;0;0;0;0;0;0;0;0;0;0;0;0;0;0;0;0;0;0;0;0;0;0;0;0;0;0;0;0;0;0;0;0;0;0;0;0;0;0;0;0;0;0;0;0;0;0;0;0;0;0;0;0;0;0;0;0;0;0;0;0;0;0;0;0] V  batteryVoltage_nominal_specify=off  batteryVoltage_nominal_value=1  batteryVoltage_nominal_unit=V  batteryCurrent_specify=on  batteryCurrent_priority=None  batteryCurrent=[0;0;0;0;0;0;0;0;0;0;0;0;0;0;0;0;0;0;0;0;0;0;0;0;0;0;0;0;0;0;0;0;0;0;0;0;0;0;0;0;0;0;0;0;0;0;0;0;0;0;0;0;0;0;0;0;0;0;0;0;0;0;0;0;0;0;0;0;0;0;0;0;0;0;0] A  batteryCurrent_nominal_specify=off  batteryCurrent_nominal_value=1  batteryCurrent_nominal_unit=A  numCycles_specify=on  numCycles_priority=High  numCycles=[0;0;0;0;0;0;0;0;0;0;0;0;0;0;0;0;0;0;0;0;0;0;0;0;0;0;0;0;0;0;0;0;0;0;0;0;0;0;0;0;0;0;0;0;0;0;0;0;0;0;0;0;0;0;0;0;0;0;0;0;0;0;0;0;0;0;0;0;0;0;0;0;0;0;0]  numCycles_nominal_specify=off  numCycles_nominal_value=1  numCycles_nominal_unit=1  vParallelAssembly_specify=on  vParallelAssembly_priority=None  vParallelAssembly=[0;0;0;0;0;0;0;0;0;0;0;0;0;0;0] V  vParallelAssembly_nominal_specify=off  vParallelAssembly_nominal_value=1  vParallelAssembly_nominal_unit=V  socParallelAssembly_specify=on  socParallelAssembly_priority=None  socParallelAssembly=[1;1;1;1;1;1;1;1;1;1;1;1;1;1;1]  socParallelAssembly_nominal_specify=off  socParallelAssembly_nominal_value=1  socParallelAssembly_nominal_unit=1
  Module5_outputs : SimscapeProbe  BoundBlock=97  Variables="{\"batteryCurrent\":{\"Probing\":\"ON\"},\"batteryVoltage\":{\"Probing\":\"ON\"},\"numCycles\":{\"Probing\":\"ON\"},\"socCell\":{\"Probing\":\"ON\"},\"socParallelAssembly\":{\"Probing\":\"ON\"},\"vParallelAssembly\":{\"Probing\":\"ON\"}}"
  Segment : Batteries_lib/Modules/ModuleType1  BatteryCapacityCell=BatteryPack.Segment.BatteryCapacityCell A*hr  ExtrapolationMethodCell=simscape.enum.extrapolation.nearest  SOCBreakpointsCell=BatteryPack.Segment.SOCBreakpointsCell  TemperatureBreakpointsCell=BatteryPack.Segment.TemperatureBreakpointsCell K  OpenCircuitVoltageThermalCell=BatteryPack.Segment.OpenCircuitVoltageThermalCell V  VoltageRangeCell=BatteryPack.Segment.VoltageRangeCell V  ResistanceSOCBreakpointsCell=BatteryPack.Segment.ResistanceSOCBreakpointsCell  ResistanceTemperatureBreakpointsCell=BatteryPack.Segment.ResistanceTemperatureBreakpointsCell K  R0ThermalCell=BatteryPack.Segment.R0ThermalCell Ohm  SimulationTemperatureCell=BatteryPack.Segment.SimulationTemperatureCell K  socCell_specify=on  socCell_priority=High  socCell=[1;1;1;1;1;1;1;1;1;1;1;1;1;1;1;1;1;1;1;1;1;1;1;1;1;1;1;1;1;1;1;1;1;1;1;1;1;1;1;1;1;1;1;1;1;1;1;1;1;1;1;1;1;1;1;1;1;1;1;1;1;1;1;1;1;1;1;1;1;1;1;1;1;1;1]  socCell_nominal_specify=off  socCell_nominal_value=1  socCell_nominal_unit=1  batteryVoltage_specify=on  batteryVoltage_priority=None  batteryVoltage=[0;0;0;0;0;0;0;0;0;0;0;0;0;0;0;0;0;0;0;0;0;0;0;0;0;0;0;0;0;0;0;0;0;0;0;0;0;0;0;0;0;0;0;0;0;0;0;0;0;0;0;0;0;0;0;0;0;0;0;0;0;0;0;0;0;0;0;0;0;0;0;0;0;0;0] V  batteryVoltage_nominal_specify=off  batteryVoltage_nominal_value=1  batteryVoltage_nominal_unit=V  batteryCurrent_specify=on  batteryCurrent_priority=None  batteryCurrent=[0;0;0;0;0;0;0;0;0;0;0;0;0;0;0;0;0;0;0;0;0;0;0;0;0;0;0;0;0;0;0;0;0;0;0;0;0;0;0;0;0;0;0;0;0;0;0;0;0;0;0;0;0;0;0;0;0;0;0;0;0;0;0;0;0;0;0;0;0;0;0;0;0;0;0] A  batteryCurrent_nominal_specify=off  batteryCurrent_nominal_value=1  batteryCurrent_nominal_unit=A  numCycles_specify=on  numCycles_priority=High  numCycles=[0;0;0;0;0;0;0;0;0;0;0;0;0;0;0;0;0;0;0;0;0;0;0;0;0;0;0;0;0;0;0;0;0;0;0;0;0;0;0;0;0;0;0;0;0;0;0;0;0;0;0;0;0;0;0;0;0;0;0;0;0;0;0;0;0;0;0;0;0;0;0;0;0;0;0]  numCycles_nominal_specify=off  numCycles_nominal_value=1  numCycles_nominal_unit=1  vParallelAssembly_specify=on  vParallelAssembly_priority=None  vParallelAssembly=[0;0;0;0;0;0;0;0;0;0;0;0;0;0;0] V  vParallelAssembly_nominal_specify=off  vParallelAssembly_nominal_value=1  vParallelAssembly_nominal_unit=V  socParallelAssembly_specify=on  socParallelAssembly_priority=None  socParallelAssembly=[1;1;1;1;1;1;1;1;1;1;1;1;1;1;1]  socParallelAssembly_nominal_specify=off  socParallelAssembly_nominal_value=1  socParallelAssembly_nominal_unit=1
  Segment_outputs : SimscapeProbe  BoundBlock=99  Variables="{\"batteryCurrent\":{\"Probing\":\"ON\"},\"batteryVoltage\":{\"Probing\":\"ON\"},\"numCycles\":{\"Probing\":\"ON\"},\"socCell\":{\"Probing\":\"ON\"},\"socParallelAssembly\":{\"Probing\":\"ON\"},\"vParallelAssembly\":{\"Probing\":\"ON\"}}"
  batteryCurrentMux : Mux  Inputs=5
  batteryVoltageMux : Mux  Inputs=5
  numCyclesMux : Mux  Inputs=5
  socCellMux : Mux  Inputs=5
  socParallelAssemblyMux : Mux  Inputs=5
  vParallelAssemblyMux : Mux  Inputs=5
  + : PMIOPort  Side=Left
  - : PMIOPort  Port=2  Side=Right
  batteryCurrent : Outport
  batteryVoltage : Outport  Port=2
  numCycles : Outport  Port=3
  socCell : Outport  Port=4
  socParallelAssembly : Outport  Port=5
  vParallelAssembly : Outport  Port=6
  wires:
  [vParallelAssembly5] -> vParallelAssemblyMux/5
  Module5_outputs/6 -> [vParallelAssembly5]
  [socParallelAssembly5] -> socParallelAssemblyMux/5
  Module5_outputs/5 -> [socParallelAssembly5]
  [socCell5] -> socCellMux/5
  Module5_outputs/4 -> [socCell5]
  [numCycles5] -> numCyclesMux/5
  Module5_outputs/3 -> [numCycles5]
  [batteryVoltage5] -> batteryVoltageMux/5
  Module5_outputs/2 -> [batteryVoltage5]
  [batteryCurrent5] -> batteryCurrentMux/5
  Module5_outputs/1 -> [batteryCurrent5]
  [vParallelAssembly4] -> vParallelAssemblyMux/4
  Module4_outputs/6 -> [vParallelAssembly4]
  [socParallelAssembly4] -> socParallelAssemblyMux/4
  Module4_outputs/5 -> [socParallelAssembly4]
  [socCell4] -> socCellMux/4
  Module4_outputs/4 -> [socCell4]
  [numCycles4] -> numCyclesMux/4
  Module4_outputs/3 -> [numCycles4]
  [batteryVoltage4] -> batteryVoltageMux/4
  Module4_outputs/2 -> [batteryVoltage4]
  [batteryCurrent4] -> batteryCurrentMux/4
  Module4_outputs/1 -> [batteryCurrent4]
  [vParallelAssembly3] -> vParallelAssemblyMux/3
  Module3_outputs/6 -> [vParallelAssembly3]
  [socParallelAssembly3] -> socParallelAssemblyMux/3
  Module3_outputs/5 -> [socParallelAssembly3]
  [socCell3] -> socCellMux/3
  Module3_outputs/4 -> [socCell3]
  [numCycles3] -> numCyclesMux/3
  Module3_outputs/3 -> [numCycles3]
  [batteryVoltage3] -> batteryVoltageMux/3
  Module3_outputs/2 -> [batteryVoltage3]
  [batteryCurrent3] -> batteryCurrentMux/3
  Module3_outputs/1 -> [batteryCurrent3]
  [vParallelAssembly2] -> vParallelAssemblyMux/2
  Module2_outputs/6 -> [vParallelAssembly2]
  [socParallelAssembly2] -> socParallelAssemblyMux/2
  Module2_outputs/5 -> [socParallelAssembly2]
  [socCell2] -> socCellMux/2
  Module2_outputs/4 -> [socCell2]
  [numCycles2] -> numCyclesMux/2
  Module2_outputs/3 -> [numCycles2]
  [batteryVoltage2] -> batteryVoltageMux/2
  Module2_outputs/2 -> [batteryVoltage2]
  [batteryCurrent2] -> batteryCurrentMux/2
  Module2_outputs/1 -> [batteryCurrent2]
  [vParallelAssembly1] -> vParallelAssemblyMux/1
  vParallelAssemblyMux/1 -> vParallelAssembly/1
  Segment_outputs/6 -> [vParallelAssembly1]
  [socParallelAssembly1] -> socParallelAssemblyMux/1
  socParallelAssemblyMux/1 -> socParallelAssembly/1
  Segment_outputs/5 -> [socParallelAssembly1]
  [socCell1] -> socCellMux/1
  socCellMux/1 -> socCell/1
  Segment_outputs/4 -> [socCell1]
  [numCycles1] -> numCyclesMux/1
  numCyclesMux/1 -> numCycles/1
  Segment_outputs/3 -> [numCycles1]
  [batteryVoltage1] -> batteryVoltageMux/1
  batteryVoltageMux/1 -> batteryVoltage/1
  Segment_outputs/2 -> [batteryVoltage1]
  [batteryCurrent1] -> batteryCurrentMux/1
  batteryCurrentMux/1 -> batteryCurrent/1
  Segment_outputs/1 -> [batteryCurrent1]
  connections:
  Module5/RConn1 -- -/RConn1
  Segment/LConn1 -- +/RConn1
  Module5/LConn1 -- Module4/RConn1
  Module4/LConn1 -- Module3/RConn1
  Module3/LConn1 -- Module2/RConn1
  Module2/LConn1 -- Segment/RConn1
